simulink model "evapSimNew"  (R2023b)
settings: Solver=ode15s  StartTime=0.0  StopTime=3000  RelTol=1e-6
libraries: slpidlib x1
settings Model: Creator=s262314  LastModifiedBy=rhandleycajote
settings SolverCC: AlgebraicLoopSolver=TrustRegion
settings DataIOCC: ReturnWorkspaceOutputs=off  OutputOption=SpecifiedOutputTimes  OutputTimes=[0:0.5:3000]
settings DebuggingCC: UnconnectedInputMsg=warning  UnconnectedOutputMsg=warning  UnconnectedLineMsg=warning  ArithmeticOperatorsInVariantConditions=warning
settings ModelReferenceCC: EnableRefExpFcnMdlSchedulingChecks=on
settings SFSimCC: SimUseLocalCustomCode=off  CustomCodeUndefinedFunction=UseInterfaceOnly
settings RTWCC: RTWUseLocalCustomCode=off
settings CodeAppCC: StateflowObjectComments=on

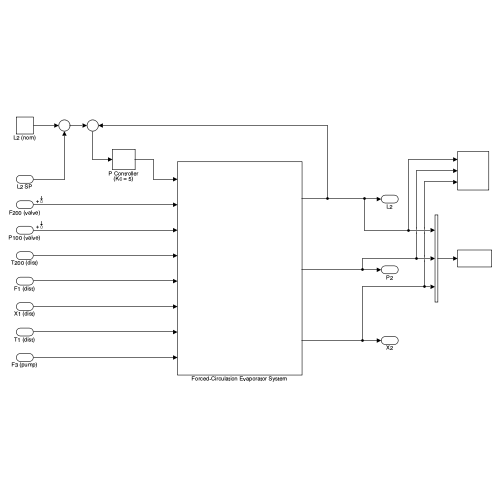
[thumbnail: Simulink's stored preview of the top-level diagram]
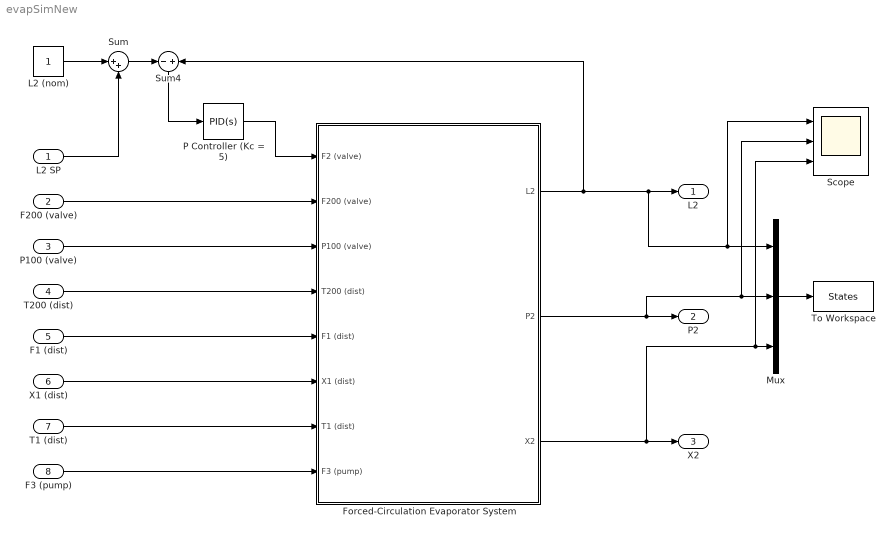
== system evapSimNew ==
  L2 SP : Inport
  F200 (valve) : Inport  Port=2
  P100 (valve) : Inport  Port=3
  T200 (dist) : Inport  Port=4
  F1 (dist) : Inport  Port=5
  X1 (dist) : Inport  Port=6
  T1 (dist) : Inport  Port=7
  F3 (pump) : Inport  Port=8
  Forced-Circulation Evaporator System : Subsystem
  L2 (nom) : Constant
  Mux : Mux  Inputs=3
  P Controller (Kc = 5) : slpidlib/PID Controller  Controller=PID  Form=Parallel  TimeDomain=Continuous-time  UseExternalTs=off  SampleTime=-1  IntegratorMethod=Forward Euler  FilterMethod=Forward Euler  ControllerParametersSource=internal  P=5  I=0  UseKiTs=off  D=0  N=100  UseFilter=on  TunerSelectOption=Transfer Function Based (PID Tuner App)  InitialConditionSource=internal  InitialConditionForIntegrator=0  InitialConditionForFilter=0  DifferentiatorICPrevScaledInput=0  ExternalReset=none  TrackingMode=off  Kt=1  LimitOutput=on  SatLimitsSource=internal  UpperSaturationLimit=2  LowerSaturationLimit=-2  LinearizeAsGain=on  AntiWindupMode=none  Kb=1  LimitIntegrator=off  UpperIntegratorSaturationLimit=inf  LowerIntegratorSaturationLimit=-inf  POutMin=[]  POutMax=[]  IOutMin=[]  IOutMax=[]  DOutMin=[]  DOutMax=[]  NOutMin=[]  NOutMax=[]  SumOutMin=[]  SumOutMax=[]  SaturationOutMin=[]  SaturationOutMax=[]  PParamMin=[]  PParamMax=[]  IParamMin=[]  IParamMax=[]  DParamMin=[]  DParamMax=[]  NParamMin=[]  NParamMax=[]  KbParamMin=[]  KbParamMax=[]  KtParamMin=[]  KtParamMax=[]  KbOutMin=[]  KbOutMax=[]  KtOutMin=[]  KtOutMax=[]  IntegratorOutMin=[]  IntegratorOutMax=[]  FilterOutMin=[]  FilterOutMax=[]  SumI1OutMin=[]  SumI1OutMax=[]  SumI2OutMin=[]  SumI2OutMax=[]  SumI3OutMin=[]  SumI3OutMax=[]  SumI4OutMin=[]  SumI4OutMax=[]  SumDOutMin=[]  SumDOutMax=[]  DifferentiatorOutMin=[]  DifferentiatorOutMax=[]  FilterDiffOutCoefMin=[]  FilterDiffOutCoefMax=[]  ReciprocalOutMin=[]  ReciprocalOutMax=[]  SumDenOutMin=[]  SumDenOutMax=[]  SumNumOutMin=[]  SumNumOutMax=[]  DivideOutMin=[]  DivideOutMax=[]  UdiffTsProdOutMin=[]  UdiffTsProdOutMax=[]  NTsProdOutMin=[]  NTsProdOutMax=[]  UintegralTsProdOutMin=[]  UintegralTsProdOutMax=[]  UngainTsProdOutMin=[]  UngainTsProdOutMax=[]  ClampingZeroOutDataTypeStr=Inherit: Inherit via back propagation  ClampingZeroOutMin=[]  ClampingZeroOutMax=[]  FilterDenConstantOutDataTypeStr=Inherit: Inherit via back propagation  FilterDenConstantOutMin=[]  FilterDenConstantOutMax=[]  PCopyOutDataTypeStr=Inherit: Inherit via back propagation  PCopyOutMin=[]  PCopyOutMax=[]  NCopyOutDataTypeStr=Inherit: Inherit via back propagation  NCopyOutMin=[]  NCopyOutMax=[]  IntegratorContinuousStateAttributes=''  IntegratorStateMustResolveToSignalObject=off  IntegratorRTWStateStorageClass=Auto  FilterContinuousStateAttributes=''  FilterStateMustResolveToSignalObject=off  FilterRTWStateStorageClass=Auto  ParallelPVariant=InternalParameters  IdealPVariant=Disabled  IVariant=InternalParameters  DVariant=InternalParameters  IntegratorVariant=Continuous  SatVariant=Enabled  AWVariant=Passthrough  PCopyVariant=Disabled  TRVariant=Disabled  FdbkBlocksVariant=Forward  IdealPFdbkVariant=Disabled  SatFdbkVariant=Disabled  DerivativeFilterVariant=ContFilter  NVariant=InternalParameters  NCopyVariant=Disabled  FilterICVariant=InternalICsFilter  IntegratorICVariant=InternalICs  ExternalResetVariant=Disabled  TRSumVariant=Passthrough  SumFdbkVariant=Disabled  SumVariant=Sum_PID  TsampFilterVariant=InternalTs  TsampNgainVariant=Passthrough  TsampIntegralVariant=Disabled_SignalSpec  ExternalSaturationOutDataTypeStr=Inherit: Same as second input
  Scope : Scope  NumInputPorts=3
  Sum : Sum  Inputs=|++
  Sum4 : Sum  Inputs=-|+
  To Workspace : ToWorkspace  VariableName=States  SampleTime=-1
  L2 : Outport  VectorParamsAs1DForOutWhenUnconnected=off
  P2 : Outport  Port=2  VectorParamsAs1DForOutWhenUnconnected=off
  X2 : Outport  Port=3  VectorParamsAs1DForOutWhenUnconnected=off
  wires:
  P100 (valve)/1 -> Forced-Circulation Evaporator System/3(P100 (valve))
  T200 (dist)/1 -> Forced-Circulation Evaporator System/4(T200 (dist))
  F1 (dist)/1 -> Forced-Circulation Evaporator System/5(F1 (dist))
  X1 (dist)/1 -> Forced-Circulation Evaporator System/6(X1 (dist))
  T1 (dist)/1 -> Forced-Circulation Evaporator System/7(T1 (dist))
  F3 (pump)/1 -> Forced-Circulation Evaporator System/8(F3 (pump))
  Forced-Circulation Evaporator System/2(P2) -> Scope/2, Mux/2, P2/1
  Forced-Circulation Evaporator System/3(X2) -> Scope/3, Mux/3, X2/1
  Sum/1 -> Sum4/1
  Sum4/1 -> P Controller (Kc = 5)/1
  L2 (nom)/1 -> Sum/1
  Forced-Circulation Evaporator System/1(L2) -> Scope/1, Mux/1, L2/1, Sum4/2
  Mux/1 -> To Workspace/1
  F200 (valve)/1 -> Forced-Circulation Evaporator System/2(F200 (valve))
  L2 SP/1 -> Sum/2
  P Controller (Kc = 5)/1 -> Forced-Circulation Evaporator System/1(F2 (valve))

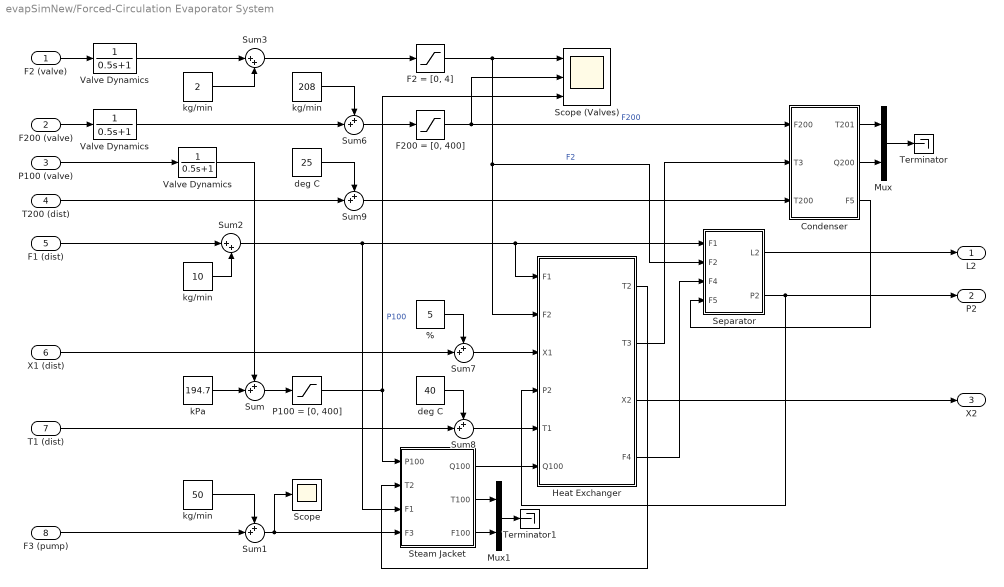
== system evapSimNew/Forced-Circulation Evaporator System ==
  F2 (valve) : Inport
  F200 (valve) : Inport  Port=2
  P100 (valve) : Inport  Port=3
  T200 (dist) : Inport  Port=4
  F1 (dist) : Inport  Port=5
  X1 (dist) : Inport  Port=6
  T1 (dist) : Inport  Port=7
  F3 (pump) : Inport  Port=8
  " Valve Dynamics" : TransferFcn  Denominator=[0.5 1]
  " deg C " : Constant  Value=25
  " kg/min" : Constant  Value=208
  " kg/min " : Constant  Value=10
  % : Constant  Value=5
  Condenser : Subsystem
  "F2 = [0, 4]" : Saturate  UpperLimit=4  LowerLimit=0  ZeroCross=off
  "F200 = [0, 400]" : Saturate  UpperLimit=400  LowerLimit=0
  Heat Exchanger : Subsystem
  Mux : Mux  Inputs=2
  Mux1 : Mux  Inputs=2
  "P100 = [0, 400]" : Saturate  UpperLimit=400  LowerLimit=0
  Scope : Scope
  Scope (Valves) : Scope  NumInputPorts=3
  Separator : Subsystem
  Steam Jacket : Subsystem
  Sum{,1,6..9} (6 alike) : Sum  Inputs=++|
  Sum2 : Sum  Inputs=|++
  Sum3 : Sum  Inputs=|++
  Terminator : Terminator
  Terminator1 : Terminator
  Valve Dynamics : TransferFcn  Denominator=[0.5 1]
  "Valve Dynamics " : TransferFcn  Denominator=[0.5 1]
  deg C : Constant  Value=40
  kPa : Constant  Value=194.7
  kg/min : Constant  Value=2
  "kg/min " : Constant  Value=50
  L2 : Outport  VectorParamsAs1DForOutWhenUnconnected=off
  P2 : Outport  Port=2  VectorParamsAs1DForOutWhenUnconnected=off
  X2 : Outport  Port=3  VectorParamsAs1DForOutWhenUnconnected=off
  wires:
  Steam Jacket/1(Q100) -> Heat Exchanger/6(Q100)
  Heat Exchanger/4(F4) -> Separator/3(F4)
  Condenser/3(F5) -> Separator/4(F5)
  Separator/2(P2) -> P2/1, Heat Exchanger/4(P2)
  Heat Exchanger/2(T3) -> Condenser/2(T3)
  Heat Exchanger/1(T2) -> Steam Jacket/2(T2)
  P100 (valve)/1 -> " Valve Dynamics"/1
  Sum/1 -> "P100 = [0, 400]"/1
  Sum1/1 -> Steam Jacket/4(F3), Scope/1
  " kg/min "/1 -> Sum2/2
  Sum2/1 -> Heat Exchanger/1(F1), Separator/1(F1), Steam Jacket/3(F1)
  "F2 = [0, 4]"/1 -> Heat Exchanger/2(F2), Separator/2(F2), Scope (Valves)/1  "F2"
  Sum6/1 -> "F200 = [0, 400]"/1
  kPa/1 -> Sum/2
  F200 (valve)/1 -> "Valve Dynamics "/1
  " kg/min"/1 -> Sum6/1
  %/1 -> Sum7/1
  Sum7/1 -> Heat Exchanger/3(X1)
  X1 (dist)/1 -> Sum7/2
  deg C/1 -> Sum8/1
  Sum8/1 -> Heat Exchanger/5(T1)
  T1 (dist)/1 -> Sum8/2
  F3 (pump)/1 -> Sum1/2
  "kg/min "/1 -> Sum1/1
  " deg C "/1 -> Sum9/1
  T200 (dist)/1 -> Sum9/2
  Mux/1 -> Terminator/1
  Condenser/1(T201) -> Mux/1
  Condenser/2(Q200) -> Mux/2
  Mux1/1 -> Terminator1/1
  Steam Jacket/3(F100) -> Mux1/2
  Steam Jacket/2(T100) -> Mux1/1
  Heat Exchanger/3(X2) -> X2/1
  "F200 = [0, 400]"/1 -> Scope (Valves)/2, Condenser/1(F200)  "F200"
  Sum9/1 -> Condenser/3(T200)
  Sum3/1 -> "F2 = [0, 4]"/1
  F2 (valve)/1 -> Valve Dynamics/1
  kg/min/1 -> Sum3/2
  "P100 = [0, 400]"/1 -> Scope (Valves)/3, Steam Jacket/1(P100)  "P100"
  Valve Dynamics/1 -> Sum3/1
  "Valve Dynamics "/1 -> Sum6/2
  " Valve Dynamics"/1 -> Sum/1
  Separator/1(L2) -> L2/1
  F1 (dist)/1 -> Sum2/1

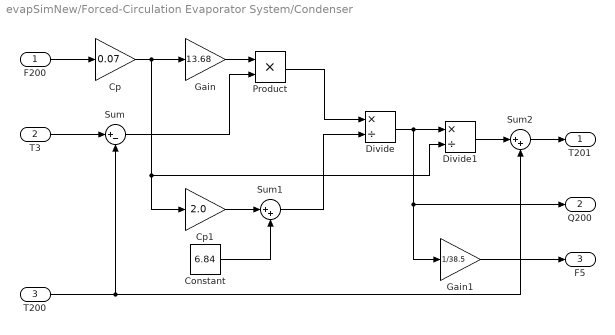
== system evapSimNew/Forced-Circulation Evaporator System/Condenser ==
  F200 : Inport
  T3 : Inport  Port=2
  T200 : Inport  Port=3
  Constant : Constant  Value=6.84
  Cp : Gain  Gain=0.07
  Cp1 : Gain  Gain=2.0
  Divide : Product  Inputs=*/
  Divide1 : Product  Inputs=*/
  Gain : Gain  Gain=13.68
  Gain1 : Gain  Gain=1/38.5
  Product : Product
  Sum : Sum  Inputs=|+-
  Sum1 : Sum  Inputs=|++
  Sum2 : Sum  Inputs=|++
  T201 : Outport  VectorParamsAs1DForOutWhenUnconnected=off
  Q200 : Outport  Port=2  VectorParamsAs1DForOutWhenUnconnected=off
  F5 : Outport  Port=3  VectorParamsAs1DForOutWhenUnconnected=off
  wires:
  T3/1 -> Sum/1
  T200/1 -> Sum/2, Sum2/2
  F200/1 -> Cp/1
  Sum/1 -> Product/2
  Cp/1 -> Cp1/1, Divide1/2, Gain/1
  Product/1 -> Divide/1
  Gain/1 -> Product/1
  Cp1/1 -> Sum1/1
  Sum1/1 -> Divide/2
  Constant/1 -> Sum1/2
  Divide/1 -> Gain1/1, Q200/1, Divide1/1
  Gain1/1 -> F5/1
  Divide1/1 -> Sum2/1
  Sum2/1 -> T201/1

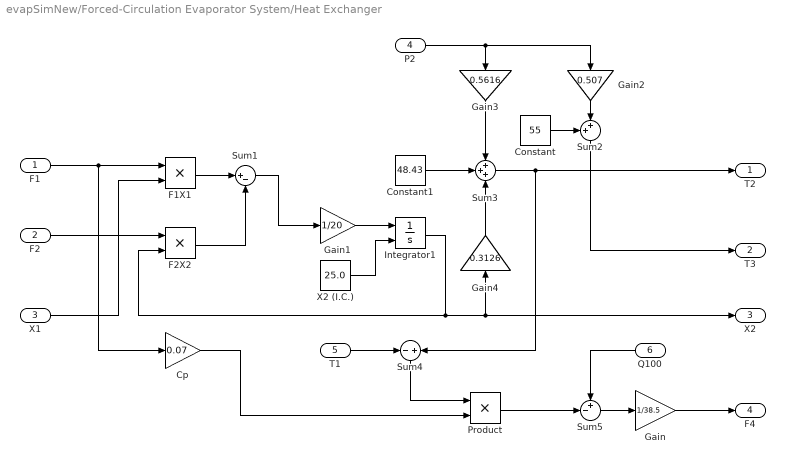
== system evapSimNew/Forced-Circulation Evaporator System/Heat Exchanger ==
  F1 : Inport
  F2 : Inport  Port=2
  X1 : Inport  Port=3
  P2 : Inport  Port=4
  T1 : Inport  Port=5
  Q100 : Inport  Port=6
  Constant : Constant  Value=55
  Constant1 : Constant  Value=48.43
  Cp : Gain  Gain=0.07
  F1X1 : Product
  F2X2 : Product
  Gain : Gain  Gain=1/38.5
  Gain1 : Gain  Gain=1/20
  Gain2 : Gain  Gain=0.507
  Gain3 : Gain  Gain=0.5616
  Gain4 : Gain  Gain=0.3126
  Integrator1 : Integrator  InitialConditionSource=external
  Product : Product
  Sum1 : Sum  Inputs=|+-
  Sum2 : Sum  Inputs=++|
  Sum3 : Sum  Inputs=+++
  Sum4 : Sum  Inputs=-|+
  Sum5 : Sum  Inputs=+-|
  X2 (I.C.) : Constant  Value=25.0
  T2 : Outport  VectorParamsAs1DForOutWhenUnconnected=off
  T3 : Outport  Port=2  VectorParamsAs1DForOutWhenUnconnected=off
  X2 : Outport  Port=3  VectorParamsAs1DForOutWhenUnconnected=off
  F4 : Outport  Port=4  VectorParamsAs1DForOutWhenUnconnected=off
  wires:
  F1/1 -> Cp/1, F1X1/1
  F2/1 -> F2X2/1
  X1/1 -> F1X1/2
  F1X1/1 -> Sum1/1
  F2X2/1 -> Sum1/2
  Sum1/1 -> Gain1/1
  Gain1/1 -> Integrator1/1
  Integrator1/1 -> X2/1, Gain4/1, F2X2/2
  X2 (I.C.)/1 -> Integrator1/2
  Gain2/1 -> Sum2/2
  Sum2/1 -> T3/1
  Constant/1 -> Sum2/1
  Gain3/1 -> Sum3/1
  Constant1/1 -> Sum3/2
  Gain4/1 -> Sum3/3
  Sum3/1 -> Sum4/2, T2/1
  P2/1 -> Gain3/1, Gain2/1
  Cp/1 -> Product/2
  T1/1 -> Sum4/1
  Sum4/1 -> Product/1
  Sum5/1 -> Gain/1
  Gain/1 -> F4/1
  Q100/1 -> Sum5/1
  Product/1 -> Sum5/2

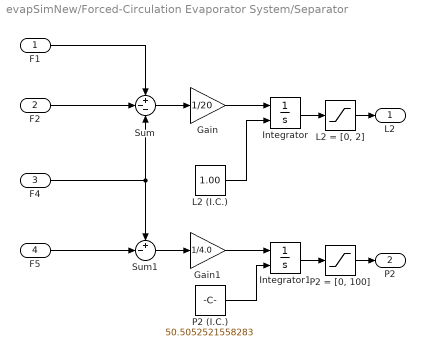
== system evapSimNew/Forced-Circulation Evaporator System/Separator ==
  F1 : Inport
  F2 : Inport  Port=2
  F4 : Inport  Port=3
  F5 : Inport  Port=4
  Gain : Gain  Gain=1/20
  Gain1 : Gain  Gain=1/4.0
  Integrator : Integrator  InitialConditionSource=external  InitialCondition=1.0
  Integrator1 : Integrator  InitialConditionSource=external
  L2 (I.C.) : Constant  Value=1.00
  "L2 = [0, 2]" : Saturate  UpperLimit=2  LowerLimit=0
  P2 (I.C.) : Constant  Value=50.5052521558283
  "P2 = [0, 100]" : Saturate  UpperLimit=100  LowerLimit=0
  Sum : Sum  Inputs=+--
  Sum1 : Sum  Inputs=+-|
  L2 : Outport  VectorParamsAs1DForOutWhenUnconnected=off
  P2 : Outport  Port=2  VectorParamsAs1DForOutWhenUnconnected=off
  wires:
  F1/1 -> Sum/1
  F2/1 -> Sum/2
  F4/1 -> Sum1/1, Sum/3
  Sum/1 -> Gain/1
  Gain/1 -> Integrator/1
  Integrator/1 -> "L2 = [0, 2]"/1
  L2 (I.C.)/1 -> Integrator/2
  Gain1/1 -> Integrator1/1
  Sum1/1 -> Gain1/1
  P2 (I.C.)/1 -> Integrator1/2
  F5/1 -> Sum1/2
  Integrator1/1 -> "P2 = [0, 100]"/1
  "P2 = [0, 100]"/1 -> P2/1
  "L2 = [0, 2]"/1 -> L2/1

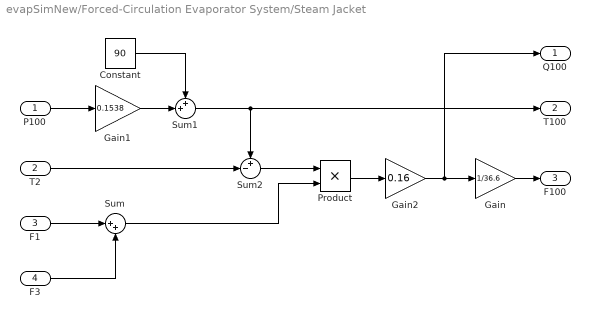
== system evapSimNew/Forced-Circulation Evaporator System/Steam Jacket ==
  P100 : Inport
  T2 : Inport  Port=2
  F1 : Inport  Port=3
  F3 : Inport  Port=4
  Constant : Constant  Value=90
  Gain : Gain  Gain=1/36.6
  Gain1 : Gain  Gain=0.1538
  Gain2 : Gain  Gain=0.16
  Product : Product
  Sum : Sum  Inputs=|++
  Sum1 : Sum  Inputs=++|
  Sum2 : Sum  Inputs=+-|
  Q100 : Outport  VectorParamsAs1DForOutWhenUnconnected=off
  T100 : Outport  Port=2  VectorParamsAs1DForOutWhenUnconnected=off
  F100 : Outport  Port=3  VectorParamsAs1DForOutWhenUnconnected=off
  wires:
  Gain/1 -> F100/1
  F1/1 -> Sum/1
  F3/1 -> Sum/2
  P100/1 -> Gain1/1
  Gain1/1 -> Sum1/2
  Constant/1 -> Sum1/1
  T2/1 -> Sum2/2
  Sum1/1 -> T100/1, Sum2/1
  Sum2/1 -> Product/1
  Sum/1 -> Product/2
  Product/1 -> Gain2/1
  Gain2/1 -> Gain/1, Q100/1
